simulink model "sistema2020_5"  (R2020b)
settings: Solver=ode15s  StartTime=0.0  StopTime=0.7  MaxStep=1E-2  RelTol=1e-3
libraries: fl_lib x20, ee_lib x12, nesl_utility x12, pid_lib x1
settings Model: LastModifiedBy=josue
settings SolverCC: AlgebraicLoopSolver=LineSearch
settings DataIOCC: SaveOutput=off  SignalLogging=off  DSMLogging=off  ReturnWorkspaceOutputs=off  TimeSaveName=t
settings DebuggingCC: AlgebraicLoopMsg=none  ArtificialAlgebraicLoopMsg=none  MaxConsecutiveZCsMsg=none  UnconnectedInputMsg=none  UnconnectedOutputMsg=none  UnconnectedLineMsg=none  ModelReferenceExtraNoncontSigs=none  OperatingPointInterfaceChecksumMismatchMsg=none
settings ModelReferenceCC: UpdateModelReferenceTargets=IfOutOfDate  EnableRefExpFcnMdlSchedulingChecks=off
settings RTWCC: GPUComputeCapability=5.0

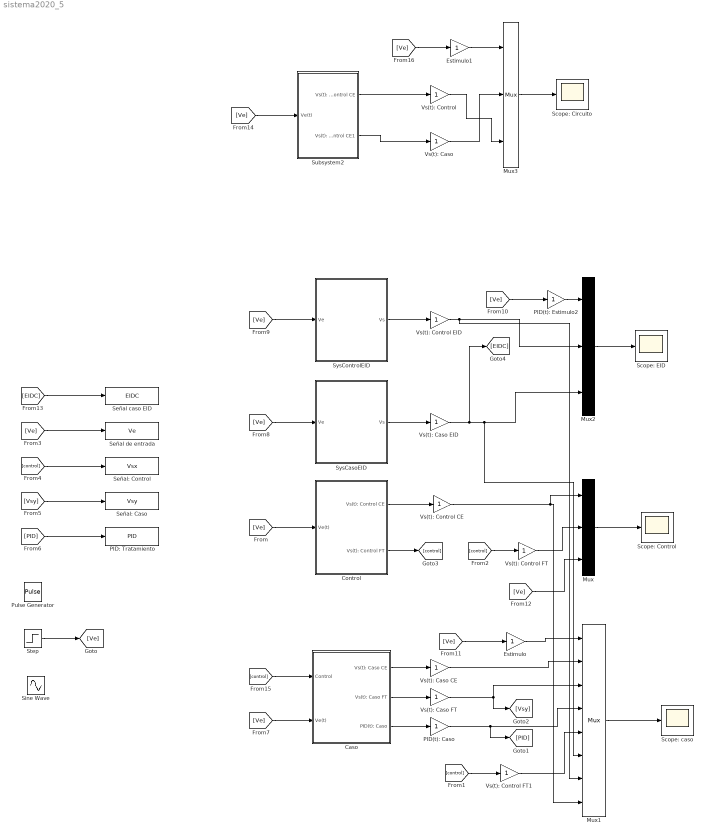
== system sistema2020_5 ==
  Caso : Subsystem
  Control : Subsystem
  Estimulo : Gain
  Estimulo1 : Gain
  Mux : Mux  Inputs=3
  Mux1 : Mux  Inputs=8
  Mux2 : Mux  Inputs=3
  Mux3 : Mux  Inputs=3
  PID(t): Caso : Gain
  PID(t): Estimulo2 : Gain
  PID: Tratamiento : ToWorkspace  VariableName=PID  SampleTime=-1
  Pulse Generator : DiscretePulseGenerator  PulseType=Time based  Period=10  PulseWidth=10  PhaseDelay=1
  Scope: Circuito : Scope
  Scope: Control : Scope
  Scope: EID : Scope
  Scope: caso : Scope
  Señal caso EID : ToWorkspace  VariableName=EIDC  SampleTime=-1
  Señal de entrada : ToWorkspace  VariableName=Ve  SampleTime=-1
  Señal: Caso : ToWorkspace  VariableName=Vsy  SampleTime=-1
  Señal: Control : ToWorkspace  VariableName=Vsx  SampleTime=-1
  Sine Wave : Sin  Frequency=pi/2
  Step : Step  Time=0  Before=1  SampleTime=0
  Subsystem2 : Subsystem
  SysCasoEID : Subsystem
  SysControlEID : Subsystem
  Vs(t): Caso : Gain
  Vs(t): Caso CE : Gain
  "Vs(t): Caso EID " : Gain
  Vs(t): Caso FT : Gain
  Vs(t): Control : Gain
  Vs(t): Control CE : Gain
  Vs(t): Control EID : Gain
  Vs(t): Control FT : Gain
  Vs(t): Control FT1 : Gain
  wires:
  Mux/1 -> Scope: Control/1
  [Ve] -> Control/1(Ve(t))
  Control/1(Vs(t): Control CE) -> Vs(t): Control CE/1
  PID(t): Caso/1 -> [PID], Mux1/4
  Vs(t): Caso CE/1 -> Mux1/2
  Vs(t): Caso FT/1 -> [Vsy], Mux1/3
  Mux1/1 -> Scope: caso/1
  Caso/1(Vs(t): Caso CE) -> Vs(t): Caso CE/1
  Caso/2(Vs(t): Caso FT) -> Vs(t): Caso FT/1
  Caso/3(PID(t): Caso) -> PID(t): Caso/1
  [Ve] -> Caso/2(Ve(t))
  [control] -> Caso/1(Control)
  [control] -> Vs(t): Control FT/1
  Control/2(Vs(t): Control FT) -> [control]
  [PID] -> PID: Tratamiento/1
  [Vsy] -> Señal: Caso/1
  [control] -> Señal: Control/1
  [Ve] -> Señal de entrada/1
  [Ve] -> SysCasoEID/1(Ve)
  Vs(t): Control CE/1 -> Mux1/8, Mux/1
  SysCasoEID/1(Vs) -> "Vs(t): Caso EID "/1
  Vs(t): Control FT/1 -> Mux/2
  [Ve] -> SysControlEID/1(Ve)
  SysControlEID/1(Vs) -> Vs(t): Control EID/1
  Mux2/1 -> Scope: EID/1
  "Vs(t): Caso EID "/1 -> [EIDC], Mux1/6, Mux2/3
  Vs(t): Control EID/1 -> Mux1/7, Mux2/2
  [Ve] -> Mux/3
  [EIDC] -> Señal caso EID/1
  [Ve] -> Subsystem2/1(Ve(t))
  Mux3/1 -> Scope: Circuito/1
  Subsystem2/1(Vs(t): Control CE) -> Vs(t): Control/1
  Subsystem2/2(Vs(t): Control CE1) -> Vs(t): Caso/1
  [Ve] -> Estimulo/1
  Estimulo1/1 -> Mux3/1
  [Ve] -> Estimulo1/1
  Step/1 -> [Ve]
  Vs(t): Caso/1 -> Mux3/2
  Vs(t): Control/1 -> Mux3/3
  [Ve] -> PID(t): Estimulo2/1
  PID(t): Estimulo2/1 -> Mux2/1
  Estimulo/1 -> Mux1/1
  [control] -> Vs(t): Control FT1/1
  Vs(t): Control FT1/1 -> Mux1/5

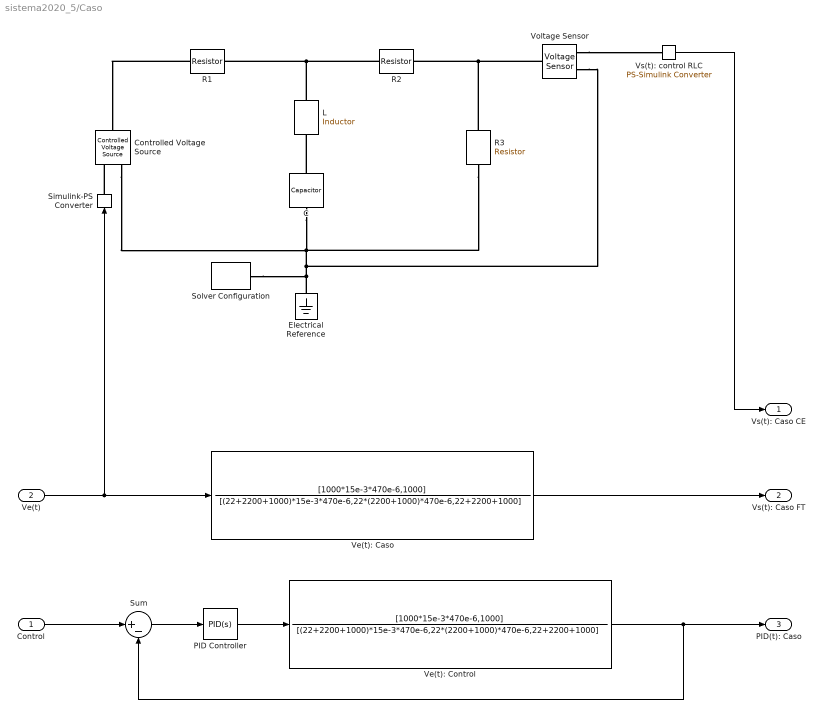
== system sistema2020_5/Caso ==
  Control : Inport
  Ve(t) : Inport  Port=2
  C : fl_lib/Electrical/Electrical Elements/Capacitor  c=470e-6 F  r=1e-6 Ohm  g=0 1/Ohm  i_specify=off  i_priority=None  i=0 A  i_nominal_specify=off  i_nominal_unit=A  i_nominal_value=1  v_specify=off  v_priority=None  v=0 V  v_nominal_specify=off  v_nominal_unit=V  v_nominal_value=1  vc_specify=off  vc_priority=High  vc=0 V  vc_nominal_specify=off  vc_nominal_unit=V  vc_nominal_value=1
  Controlled Voltage Source : fl_lib/Electrical/Electrical Sources/Controlled Voltage Source
  Electrical Reference : fl_lib/Electrical/Electrical Elements/Electrical Reference
  L : fl_lib/Electrical/Electrical Elements/Inductor  l=15e-3 H  r=0 Ohm  g=1e-9 1/Ohm  i_specify=off  i_priority=None  i=0 A  i_nominal_specify=off  i_nominal_unit=A  i_nominal_value=1  v_specify=off  v_priority=None  v=0 V  v_nominal_specify=off  v_nominal_unit=V  v_nominal_value=1  i_L_specify=off  i_L_priority=High  i_L=0 A  i_L_nominal_specify=off  i_L_nominal_unit=A  i_L_nominal_value=1
  PID Controller : pid_lib/PID Controller  Controller=PID  Form=Parallel  TimeDomain=Continuous-time  UseExternalTs=off  SampleTime=-1  IntegratorMethod=Forward Euler  FilterMethod=Forward Euler  ControllerParametersSource=internal  P=34.7718893350657  I=7760.09166130788  D=0.0231467186485559  UseFilter=on  N=113714.226471801  TunerSelectOption=Transfer Function Based (PID Tuner App)  InitialConditionSource=internal  InitialConditionForIntegrator=0  InitialConditionForFilter=0  DifferentiatorICPrevScaledInput=0  ExternalReset=none  TrackingMode=off  Kt=1  LimitOutput=off  SatLimitsSource=internal  UpperSaturationLimit=inf  LowerSaturationLimit=-inf  LinearizeAsGain=on  AntiWindupMode=none  Kb=1  POutMin=[]  POutMax=[]  IOutMin=[]  IOutMax=[]  DOutMin=[]  DOutMax=[]  NOutMin=[]  NOutMax=[]  SumOutMin=[]  SumOutMax=[]  SaturationOutMin=[]  SaturationOutMax=[]  PParamMin=[]  PParamMax=[]  IParamMin=[]  IParamMax=[]  DParamMin=[]  DParamMax=[]  NParamMin=[]  NParamMax=[]  KbParamMin=[]  KbParamMax=[]  KtParamMin=[]  KtParamMax=[]  KbOutMin=[]  KbOutMax=[]  KtOutMin=[]  KtOutMax=[]  IntegratorOutMin=[]  IntegratorOutMax=[]  FilterOutMin=[]  FilterOutMax=[]  SumI1OutMin=[]  SumI1OutMax=[]  SumI2OutMin=[]  SumI2OutMax=[]  SumI3OutMin=[]  SumI3OutMax=[]  SumI4OutMin=[]  SumI4OutMax=[]  SumDOutMin=[]  SumDOutMax=[]  DifferentiatorOutMin=[]  DifferentiatorOutMax=[]  FilterDiffOutCoefMin=[]  FilterDiffOutCoefMax=[]  ReciprocalOutMin=[]  ReciprocalOutMax=[]  SumDenOutMin=[]  SumDenOutMax=[]  SumNumOutMin=[]  SumNumOutMax=[]  DivideOutMin=[]  DivideOutMax=[]  UdiffTsProdOutMin=[]  UdiffTsProdOutMax=[]  NTsProdOutMin=[]  NTsProdOutMax=[]  UintegralTsProdOutMin=[]  UintegralTsProdOutMax=[]  UngainTsProdOutMin=[]  UngainTsProdOutMax=[]  IntegratorContinuousStateAttributes=''  IntegratorStateMustResolveToSignalObject=off  IntegratorRTWStateStorageClass=Auto  FilterContinuousStateAttributes=''  FilterStateMustResolveToSignalObject=off  FilterRTWStateStorageClass=Auto  ParallelPVariant=InternalParameters  IdealPVariant=Disabled  IVariant=InternalParameters  DVariant=InternalParameters  IntegratorVariant=Continuous  SatVariant=Disabled  AWVariant=Passthrough  PCopyVariant=Disabled  TRVariant=Disabled  FdbkBlocksVariant=Forward  IdealPFdbkVariant=Disabled  SatFdbkVariant=Disabled  DerivativeFilterVariant=ContFilter  NVariant=InternalParameters  NCopyVariant=Disabled  FilterICVariant=InternalICsFilter  IntegratorICVariant=InternalICs  ExternalResetVariant=Disabled  TRSumVariant=Passthrough  SumFdbkVariant=Disabled  SumVariant=Sum_PID  TsampFilterVariant=InternalTs  TsampNgainVariant=Passthrough  TsampIntegralVariant=Passthrough  ExternalSaturationOutDataTypeStr=Inherit: Same as second input
  R1 : ee_lib/Passive/Resistor  R=22 Ohm  R_tol=5  enable_R_tol=0  tol_distribution=1  nSigma=4  enable_operating_limits=0  operating_limit_action=2  max_working_voltage=100 V  power_rating=1 W  enable_faults=0  fault_action=1  R_faulted=inf Ohm  enable_temporal_fault=0  t_fault=1 s  enable_behavioral_fault=0  max_permissible_current=1 A  t_fail_on_current=1 s  noise_mode=0  sample_time=1e-3 s  repeatability=1  auto_seed=2645891737  user_seed=0  Tdevice=25 degC  alpha=3.93e-3 1/K  Tmeas=25 degC  thermal_mass=100 J/K  power_derating_T1=70 degC  power_derating_T2=155 degC  operating_temperature_range_vec=[-50, 150] degC  temperature_specify=off  temperature_priority=High  temperature=298.15 K  temperature_nominal_specify=off  temperature_nominal_unit=K  temperature_nominal_value=1
  R2 : ee_lib/Passive/Resistor  R=2200 Ohm  R_tol=5  enable_R_tol=0  tol_distribution=1  nSigma=4  enable_operating_limits=0  operating_limit_action=2  max_working_voltage=100 V  power_rating=1 W  enable_faults=0  fault_action=1  R_faulted=inf Ohm  enable_temporal_fault=0  t_fault=1 s  enable_behavioral_fault=0  max_permissible_current=1 A  t_fail_on_current=1 s  noise_mode=0  sample_time=1e-3 s  repeatability=1  auto_seed=2032760128  user_seed=0  Tdevice=25 degC  alpha=3.93e-3 1/K  Tmeas=25 degC  thermal_mass=100 J/K  power_derating_T1=70 degC  power_derating_T2=155 degC  operating_temperature_range_vec=[-50, 150] degC  temperature_specify=off  temperature_priority=High  temperature=298.15 K  temperature_nominal_specify=off  temperature_nominal_unit=K  temperature_nominal_value=1
  R3 : ee_lib/Passive/Resistor  R=1000 Ohm  R_tol=5  enable_R_tol=0  tol_distribution=1  nSigma=4  enable_operating_limits=0  operating_limit_action=2  max_working_voltage=100 V  power_rating=1 W  enable_faults=0  fault_action=1  R_faulted=inf Ohm  enable_temporal_fault=0  t_fault=1 s  enable_behavioral_fault=0  max_permissible_current=1 A  t_fail_on_current=1 s  noise_mode=0  sample_time=1e-3 s  repeatability=1  auto_seed=1510366082  user_seed=0  Tdevice=25 degC  alpha=3.93e-3 1/K  Tmeas=25 degC  thermal_mass=100 J/K  power_derating_T1=70 degC  power_derating_T2=155 degC  operating_temperature_range_vec=[-50, 150] degC  temperature_specify=off  temperature_priority=High  temperature=298.15 K  temperature_nominal_specify=off  temperature_nominal_unit=K  temperature_nominal_value=1
  Simulink-PS Converter : nesl_utility/Simulink-PS Converter  PhysicalDomain=network_engine_domain  SubClassName=ps_input  LeftPortType=input  RightPortType=output  PseudoPeriodic=off  Frequencies=[]  NoiseDistribution=none  NoiseParameters=[]  Unit=1  AffineConversion=off  FilteringAndDerivatives=provide  SimscapeFilterOrder=1  InputFilterTimeConstant=0.001  UdotUserProvided=0
  Solver Configuration : nesl_utility/Solver Configuration  PhysicalDomain=network_engine_domain  SubClassName=solver  LeftPortType=input  RightPortType=generic  Tones=[]  Harmonics=[]  SimulateNoise=off  Profile=off  UseLocalSampling=off  EnableSwitchedLinearOptims=on  FrequencyDomain=off  UseCCode=off  RelTol=0.001  AbsTol=1e-06  MinStep=1e-09  ToWorkspace=off  RevertToSquareIcSolve=off  NumHomotopyIterations=100  PhasorMode=off  PhasorModeNumHarmonics=1  DoDC=off  ResidualTolerance=1e-09  UseLocalSolver=off  LocalSolverChoice=NE_BACKWARD_EULER_ADVANCER  LocalSolverSampleTime=0.001  DoFixedCost=off  MaxNonlinIter=3  MaxModeIter=2  ComputeImpulses=off  ImpulseIterations=2  LinearAlgebra=auto  EquationFormulation=NE_TIME_EF  DelaysMemoryBudget=1024  AutomaticFiltering=on  FilteringTimeConstant=0.001  PartitionStorageMethod=AS_NEEDED  PartitionMemoryBudget=1024  PartitionMethod=ROBUST
  Sum : Sum  Inputs=|+-
  Ve(t): Caso : TransferFcn  Numerator=[1000*15e-3*470e-6,1000]  Denominator=[(22+2200+1000)*15e-3*470e-6,22*(2200+1000)*470e-6,22+2200+1000]
  Ve(t): Control : TransferFcn  Numerator=[1000*15e-3*470e-6,1000]  Denominator=[(22+2200+1000)*15e-3*470e-6,22*(2200+1000)*470e-6,22+2200+1000]
  Voltage Sensor : fl_lib/Electrical/Electrical Sensors/Voltage Sensor
  "Vs(t): control RLC " : nesl_utility/PS-Simulink Converter  PhysicalDomain=network_engine_domain  SubClassName=ps_output  LeftPortType=input  RightPortType=output  PseudoPeriodic=off  Frequencies=[]  Unit=inherit  AffineConversion=off
  Vs(t): Caso CE : Outport
  Vs(t): Caso FT : Outport  Port=2
  PID(t): Caso : Outport  Port=3
  wires:
  Sum/1 -> PID Controller/1
  PID Controller/1 -> Ve(t): Control/1
  Control/1 -> Sum/1
  Ve(t): Control/1 -> Sum/2, PID(t): Caso/1
  "Vs(t): control RLC "/1 -> Vs(t): Caso CE/1
  Ve(t): Caso/1 -> Vs(t): Caso FT/1
  Ve(t)/1 -> Ve(t): Caso/1, Simulink-PS Converter/1
  connections:
  C/RConn1 -- Voltage Sensor/RConn2 -- Solver Configuration/RConn1 -- Electrical Reference/LConn1 -- R3/RConn1 -- Controlled Voltage Source/RConn2
  R1/RConn1 -- R2/LConn1 -- L/LConn1
  Voltage Sensor/LConn1 -- R3/LConn1 -- R2/RConn1
  Voltage Sensor/RConn1 -- "Vs(t): control RLC "/LConn1
  C/LConn1 -- L/RConn1
  Simulink-PS Converter/RConn1 -- Controlled Voltage Source/RConn1
  R1/LConn1 -- Controlled Voltage Source/LConn1

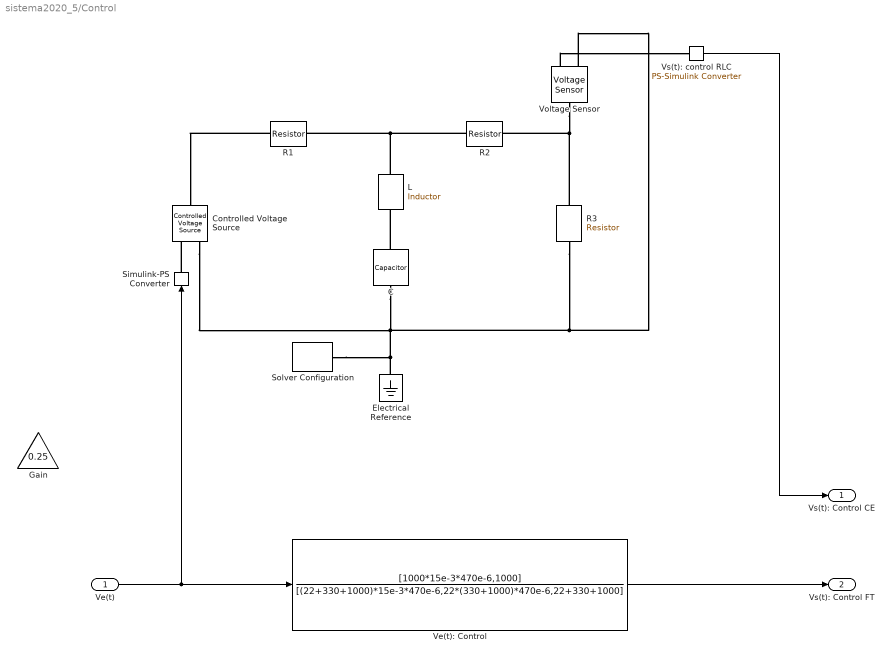
== system sistema2020_5/Control ==
  Ve(t) : Inport
  C : fl_lib/Electrical/Electrical Elements/Capacitor  c=470e-6 F  r=1e-6 Ohm  g=0 1/Ohm  i_specify=off  i_priority=None  i=0 A  i_nominal_specify=off  i_nominal_unit=A  i_nominal_value=1  v_specify=off  v_priority=None  v=0 V  v_nominal_specify=off  v_nominal_unit=V  v_nominal_value=1  vc_specify=off  vc_priority=High  vc=0 V  vc_nominal_specify=off  vc_nominal_unit=V  vc_nominal_value=1
  Controlled Voltage Source : fl_lib/Electrical/Electrical Sources/Controlled Voltage Source
  Electrical Reference : fl_lib/Electrical/Electrical Elements/Electrical Reference
  Gain : Gain  Gain=0.25
  L : fl_lib/Electrical/Electrical Elements/Inductor  l=15e-3 H  r=0 Ohm  g=1e-9 1/Ohm  i_specify=off  i_priority=None  i=0 A  i_nominal_specify=off  i_nominal_unit=A  i_nominal_value=1  v_specify=off  v_priority=None  v=0 V  v_nominal_specify=off  v_nominal_unit=V  v_nominal_value=1  i_L_specify=off  i_L_priority=High  i_L=0 A  i_L_nominal_specify=off  i_L_nominal_unit=A  i_L_nominal_value=1
  R1 : ee_lib/Passive/Resistor  R=22 Ohm  R_tol=5  enable_R_tol=0  tol_distribution=1  nSigma=4  enable_operating_limits=0  operating_limit_action=2  max_working_voltage=100 V  power_rating=1 W  enable_faults=0  fault_action=1  R_faulted=inf Ohm  enable_temporal_fault=0  t_fault=1 s  enable_behavioral_fault=0  max_permissible_current=1 A  t_fail_on_current=1 s  noise_mode=0  sample_time=1e-3 s  repeatability=1  auto_seed=1196140742  user_seed=0  Tdevice=25 degC  alpha=3.93e-3 1/K  Tmeas=25 degC  thermal_mass=100 J/K  power_derating_T1=70 degC  power_derating_T2=155 degC  operating_temperature_range_vec=[-50, 150] degC  temperature_specify=off  temperature_priority=High  temperature=298.15 K  temperature_nominal_specify=off  temperature_nominal_unit=K  temperature_nominal_value=1
  R2 : ee_lib/Passive/Resistor  R=330 Ohm  R_tol=5  enable_R_tol=0  tol_distribution=1  nSigma=4  enable_operating_limits=0  operating_limit_action=2  max_working_voltage=100 V  power_rating=1 W  enable_faults=0  fault_action=1  R_faulted=inf Ohm  enable_temporal_fault=0  t_fault=1 s  enable_behavioral_fault=0  max_permissible_current=1 A  t_fail_on_current=1 s  noise_mode=0  sample_time=1e-3 s  repeatability=1  auto_seed=2348838240  user_seed=0  Tdevice=25 degC  alpha=3.93e-3 1/K  Tmeas=25 degC  thermal_mass=100 J/K  power_derating_T1=70 degC  power_derating_T2=155 degC  operating_temperature_range_vec=[-50, 150] degC  temperature_specify=off  temperature_priority=High  temperature=298.15 K  temperature_nominal_specify=off  temperature_nominal_unit=K  temperature_nominal_value=1
  R3 : ee_lib/Passive/Resistor  R=1000 Ohm  R_tol=5  enable_R_tol=0  tol_distribution=1  nSigma=4  enable_operating_limits=0  operating_limit_action=2  max_working_voltage=100 V  power_rating=1 W  enable_faults=0  fault_action=1  R_faulted=inf Ohm  enable_temporal_fault=0  t_fault=1 s  enable_behavioral_fault=0  max_permissible_current=1 A  t_fail_on_current=1 s  noise_mode=0  sample_time=1e-3 s  repeatability=1  auto_seed=4112460543  user_seed=0  Tdevice=25 degC  alpha=3.93e-3 1/K  Tmeas=25 degC  thermal_mass=100 J/K  power_derating_T1=70 degC  power_derating_T2=155 degC  operating_temperature_range_vec=[-50, 150] degC  temperature_specify=off  temperature_priority=High  temperature=298.15 K  temperature_nominal_specify=off  temperature_nominal_unit=K  temperature_nominal_value=1
  Simulink-PS Converter : nesl_utility/Simulink-PS Converter  PhysicalDomain=network_engine_domain  SubClassName=ps_input  LeftPortType=input  RightPortType=output  PseudoPeriodic=off  Frequencies=[]  NoiseDistribution=none  NoiseParameters=[]  Unit=1  AffineConversion=off  FilteringAndDerivatives=provide  SimscapeFilterOrder=1  InputFilterTimeConstant=0.001  UdotUserProvided=0
  Solver Configuration : nesl_utility/Solver Configuration  PhysicalDomain=network_engine_domain  SubClassName=solver  LeftPortType=input  RightPortType=generic  Tones=[]  Harmonics=[]  SimulateNoise=off  Profile=off  UseLocalSampling=off  EnableSwitchedLinearOptims=on  FrequencyDomain=off  UseCCode=off  RelTol=0.001  AbsTol=1e-06  MinStep=1e-09  ToWorkspace=off  RevertToSquareIcSolve=off  NumHomotopyIterations=100  PhasorMode=off  PhasorModeNumHarmonics=1  DoDC=off  ResidualTolerance=1e-09  UseLocalSolver=off  LocalSolverChoice=NE_BACKWARD_EULER_ADVANCER  LocalSolverSampleTime=0.001  DoFixedCost=off  MaxNonlinIter=3  MaxModeIter=2  ComputeImpulses=off  ImpulseIterations=2  LinearAlgebra=auto  EquationFormulation=NE_TIME_EF  DelaysMemoryBudget=1024  AutomaticFiltering=on  FilteringTimeConstant=0.001  PartitionStorageMethod=AS_NEEDED  PartitionMemoryBudget=1024  PartitionMethod=ROBUST
  Ve(t): Control : TransferFcn  Numerator=[1000*15e-3*470e-6,1000]  Denominator=[(22+330+1000)*15e-3*470e-6,22*(330+1000)*470e-6,22+330+1000]
  Voltage Sensor : fl_lib/Electrical/Electrical Sensors/Voltage Sensor
  "Vs(t): control RLC " : nesl_utility/PS-Simulink Converter  PhysicalDomain=network_engine_domain  SubClassName=ps_output  LeftPortType=input  RightPortType=output  PseudoPeriodic=off  Frequencies=[]  Unit=inherit  AffineConversion=off
  Vs(t): Control CE : Outport
  Vs(t): Control FT : Outport  Port=2
  wires:
  Ve(t): Control/1 -> Vs(t): Control FT/1
  Ve(t)/1 -> Ve(t): Control/1, Simulink-PS Converter/1
  "Vs(t): control RLC "/1 -> Vs(t): Control CE/1
  connections:
  Voltage Sensor/LConn1 -- R3/LConn1 -- R2/RConn1
  C/RConn1 -- Voltage Sensor/RConn2 -- R3/RConn1 -- Controlled Voltage Source/RConn2 -- Solver Configuration/RConn1 -- Electrical Reference/LConn1
  R1/RConn1 -- R2/LConn1 -- L/LConn1
  Simulink-PS Converter/RConn1 -- Controlled Voltage Source/RConn1
  R1/LConn1 -- Controlled Voltage Source/LConn1
  Voltage Sensor/RConn1 -- "Vs(t): control RLC "/LConn1
  C/LConn1 -- L/RConn1

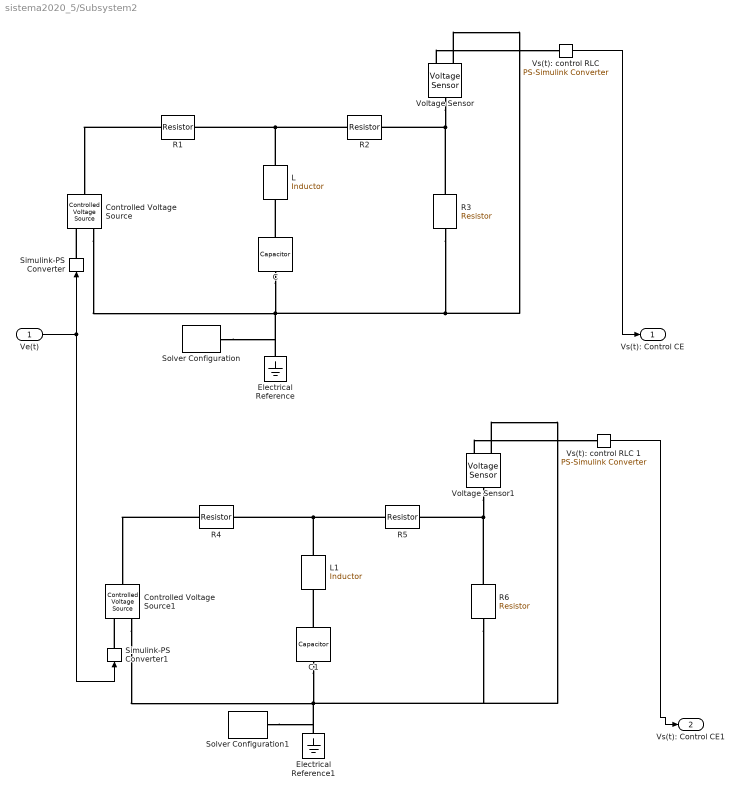
== system sistema2020_5/Subsystem2 ==
  Ve(t) : Inport
  C : fl_lib/Electrical/Electrical Elements/Capacitor  c=470e-6 F  r=1e-6 Ohm  g=0 1/Ohm  i_specify=off  i_priority=None  i=0 A  i_nominal_specify=off  i_nominal_unit=A  i_nominal_value=1  v_specify=off  v_priority=None  v=0 V  v_nominal_specify=off  v_nominal_unit=V  v_nominal_value=1  vc_specify=off  vc_priority=High  vc=0 V  vc_nominal_specify=off  vc_nominal_unit=V  vc_nominal_value=1
  C1 : fl_lib/Electrical/Electrical Elements/Capacitor  c=470e-6 F  r=1e-6 Ohm  g=0 1/Ohm  i_specify=off  i_priority=None  i=0 A  i_nominal_specify=off  i_nominal_unit=A  i_nominal_value=1  v_specify=off  v_priority=None  v=0 V  v_nominal_specify=off  v_nominal_unit=V  v_nominal_value=1  vc_specify=off  vc_priority=High  vc=0 V  vc_nominal_specify=off  vc_nominal_unit=V  vc_nominal_value=1
  Controlled Voltage Source : fl_lib/Electrical/Electrical Sources/Controlled Voltage Source
  Controlled Voltage Source1 : fl_lib/Electrical/Electrical Sources/Controlled Voltage Source
  Electrical Reference : fl_lib/Electrical/Electrical Elements/Electrical Reference
  Electrical Reference1 : fl_lib/Electrical/Electrical Elements/Electrical Reference
  L : fl_lib/Electrical/Electrical Elements/Inductor  l=15e-3 H  r=0 Ohm  g=1e-9 1/Ohm  i_specify=off  i_priority=None  i=0 A  i_nominal_specify=off  i_nominal_unit=A  i_nominal_value=1  v_specify=off  v_priority=None  v=0 V  v_nominal_specify=off  v_nominal_unit=V  v_nominal_value=1  i_L_specify=off  i_L_priority=High  i_L=0 A  i_L_nominal_specify=off  i_L_nominal_unit=A  i_L_nominal_value=1
  L1 : fl_lib/Electrical/Electrical Elements/Inductor  l=15e-3 H  r=0 Ohm  g=1e-9 1/Ohm  i_specify=off  i_priority=None  i=0 A  i_nominal_specify=off  i_nominal_unit=A  i_nominal_value=1  v_specify=off  v_priority=None  v=0 V  v_nominal_specify=off  v_nominal_unit=V  v_nominal_value=1  i_L_specify=off  i_L_priority=High  i_L=0 A  i_L_nominal_specify=off  i_L_nominal_unit=A  i_L_nominal_value=1
  R1 : ee_lib/Passive/Resistor  R=22 Ohm  R_tol=5  enable_R_tol=0  tol_distribution=1  nSigma=4  enable_operating_limits=0  operating_limit_action=2  max_working_voltage=100 V  power_rating=1 W  enable_faults=0  fault_action=1  R_faulted=inf Ohm  enable_temporal_fault=0  t_fault=1 s  enable_behavioral_fault=0  max_permissible_current=1 A  t_fail_on_current=1 s  noise_mode=0  sample_time=1e-3 s  repeatability=1  auto_seed=386335224  user_seed=0  Tdevice=25 degC  alpha=3.93e-3 1/K  Tmeas=25 degC  thermal_mass=100 J/K  power_derating_T1=70 degC  power_derating_T2=155 degC  operating_temperature_range_vec=[-50, 150] degC  temperature_specify=off  temperature_priority=High  temperature=298.15 K  temperature_nominal_specify=off  temperature_nominal_unit=K  temperature_nominal_value=1
  R2 : ee_lib/Passive/Resistor  R=330 Ohm  R_tol=5  enable_R_tol=0  tol_distribution=1  nSigma=4  enable_operating_limits=0  operating_limit_action=2  max_working_voltage=100 V  power_rating=1 W  enable_faults=0  fault_action=1  R_faulted=inf Ohm  enable_temporal_fault=0  t_fault=1 s  enable_behavioral_fault=0  max_permissible_current=1 A  t_fail_on_current=1 s  noise_mode=0  sample_time=1e-3 s  repeatability=1  auto_seed=3499211588  user_seed=0  Tdevice=25 degC  alpha=3.93e-3 1/K  Tmeas=25 degC  thermal_mass=100 J/K  power_derating_T1=70 degC  power_derating_T2=155 degC  operating_temperature_range_vec=[-50, 150] degC  temperature_specify=off  temperature_priority=High  temperature=298.15 K  temperature_nominal_specify=off  temperature_nominal_unit=K  temperature_nominal_value=1
  R3 : ee_lib/Passive/Resistor  R=1000 Ohm  R_tol=5  enable_R_tol=0  tol_distribution=1  nSigma=4  enable_operating_limits=0  operating_limit_action=2  max_working_voltage=100 V  power_rating=1 W  enable_faults=0  fault_action=1  R_faulted=inf Ohm  enable_temporal_fault=0  t_fault=1 s  enable_behavioral_fault=0  max_permissible_current=1 A  t_fail_on_current=1 s  noise_mode=0  sample_time=1e-3 s  repeatability=1  auto_seed=1943870165  user_seed=0  Tdevice=25 degC  alpha=3.93e-3 1/K  Tmeas=25 degC  thermal_mass=100 J/K  power_derating_T1=70 degC  power_derating_T2=155 degC  operating_temperature_range_vec=[-50, 150] degC  temperature_specify=off  temperature_priority=High  temperature=298.15 K  temperature_nominal_specify=off  temperature_nominal_unit=K  temperature_nominal_value=1
  R4 : ee_lib/Passive/Resistor  R=22 Ohm  R_tol=5  enable_R_tol=0  tol_distribution=1  nSigma=4  enable_operating_limits=0  operating_limit_action=2  max_working_voltage=100 V  power_rating=1 W  enable_faults=0  fault_action=1  R_faulted=inf Ohm  enable_temporal_fault=0  t_fault=1 s  enable_behavioral_fault=0  max_permissible_current=1 A  t_fail_on_current=1 s  noise_mode=0  sample_time=1e-3 s  repeatability=1  auto_seed=2874086048  user_seed=0  Tdevice=25 degC  alpha=3.93e-3 1/K  Tmeas=25 degC  thermal_mass=100 J/K  power_derating_T1=70 degC  power_derating_T2=155 degC  operating_temperature_range_vec=[-50, 150] degC  temperature_specify=off  temperature_priority=High  temperature=298.15 K  temperature_nominal_specify=off  temperature_nominal_unit=K  temperature_nominal_value=1
  R5 : ee_lib/Passive/Resistor  R=3300 Ohm  R_tol=5  enable_R_tol=0  tol_distribution=1  nSigma=4  enable_operating_limits=0  operating_limit_action=2  max_working_voltage=100 V  power_rating=1 W  enable_faults=0  fault_action=1  R_faulted=inf Ohm  enable_temporal_fault=0  t_fault=1 s  enable_behavioral_fault=0  max_permissible_current=1 A  t_fail_on_current=1 s  noise_mode=0  sample_time=1e-3 s  repeatability=1  auto_seed=817904655  user_seed=0  Tdevice=25 degC  alpha=3.93e-3 1/K  Tmeas=25 degC  thermal_mass=100 J/K  power_derating_T1=70 degC  power_derating_T2=155 degC  operating_temperature_range_vec=[-50, 150] degC  temperature_specify=off  temperature_priority=High  temperature=298.15 K  temperature_nominal_specify=off  temperature_nominal_unit=K  temperature_nominal_value=1
  R6 : ee_lib/Passive/Resistor  R=1000 Ohm  R_tol=5  enable_R_tol=0  tol_distribution=1  nSigma=4  enable_operating_limits=0  operating_limit_action=2  max_working_voltage=100 V  power_rating=1 W  enable_faults=0  fault_action=1  R_faulted=inf Ohm  enable_temporal_fault=0  t_fault=1 s  enable_behavioral_fault=0  max_permissible_current=1 A  t_fail_on_current=1 s  noise_mode=0  sample_time=1e-3 s  repeatability=1  auto_seed=1584484500  user_seed=0  Tdevice=25 degC  alpha=3.93e-3 1/K  Tmeas=25 degC  thermal_mass=100 J/K  power_derating_T1=70 degC  power_derating_T2=155 degC  operating_temperature_range_vec=[-50, 150] degC  temperature_specify=off  temperature_priority=High  temperature=298.15 K  temperature_nominal_specify=off  temperature_nominal_unit=K  temperature_nominal_value=1
  Simulink-PS Converter : nesl_utility/Simulink-PS Converter  PhysicalDomain=network_engine_domain  SubClassName=ps_input  LeftPortType=input  RightPortType=output  PseudoPeriodic=off  Frequencies=[]  NoiseDistribution=none  NoiseParameters=[]  Unit=1  AffineConversion=off  FilteringAndDerivatives=provide  SimscapeFilterOrder=1  InputFilterTimeConstant=0.001  UdotUserProvided=0
  Simulink-PS Converter1 : nesl_utility/Simulink-PS Converter  PhysicalDomain=network_engine_domain  SubClassName=ps_input  LeftPortType=input  RightPortType=output  PseudoPeriodic=off  Frequencies=[]  NoiseDistribution=none  NoiseParameters=[]  Unit=1  AffineConversion=off  FilteringAndDerivatives=provide  SimscapeFilterOrder=1  InputFilterTimeConstant=0.001  UdotUserProvided=0
  Solver Configuration : nesl_utility/Solver Configuration  PhysicalDomain=network_engine_domain  SubClassName=solver  LeftPortType=input  RightPortType=generic  Tones=[]  Harmonics=[]  SimulateNoise=off  Profile=off  UseLocalSampling=off  EnableSwitchedLinearOptims=on  FrequencyDomain=off  UseCCode=off  RelTol=0.001  AbsTol=1e-06  MinStep=1e-09  ToWorkspace=off  RevertToSquareIcSolve=off  NumHomotopyIterations=100  PhasorMode=off  PhasorModeNumHarmonics=1  DoDC=off  ResidualTolerance=1e-09  UseLocalSolver=off  LocalSolverChoice=NE_BACKWARD_EULER_ADVANCER  LocalSolverSampleTime=0.001  DoFixedCost=off  MaxNonlinIter=3  MaxModeIter=2  ComputeImpulses=off  ImpulseIterations=2  LinearAlgebra=auto  EquationFormulation=NE_TIME_EF  DelaysMemoryBudget=1024  AutomaticFiltering=on  FilteringTimeConstant=0.001  PartitionStorageMethod=AS_NEEDED  PartitionMemoryBudget=1024  PartitionMethod=ROBUST
  Solver Configuration1 : nesl_utility/Solver Configuration  PhysicalDomain=network_engine_domain  SubClassName=solver  LeftPortType=input  RightPortType=generic  Tones=[]  Harmonics=[]  SimulateNoise=off  Profile=off  UseLocalSampling=off  EnableSwitchedLinearOptims=on  FrequencyDomain=off  UseCCode=off  RelTol=0.001  AbsTol=1e-06  MinStep=1e-09  ToWorkspace=off  RevertToSquareIcSolve=off  NumHomotopyIterations=100  PhasorMode=off  PhasorModeNumHarmonics=1  DoDC=off  ResidualTolerance=1e-09  UseLocalSolver=off  LocalSolverChoice=NE_BACKWARD_EULER_ADVANCER  LocalSolverSampleTime=0.001  DoFixedCost=off  MaxNonlinIter=3  MaxModeIter=2  ComputeImpulses=off  ImpulseIterations=2  LinearAlgebra=auto  EquationFormulation=NE_TIME_EF  DelaysMemoryBudget=1024  AutomaticFiltering=on  FilteringTimeConstant=0.001  PartitionStorageMethod=AS_NEEDED  PartitionMemoryBudget=1024  PartitionMethod=ROBUST
  Voltage Sensor : fl_lib/Electrical/Electrical Sensors/Voltage Sensor
  Voltage Sensor1 : fl_lib/Electrical/Electrical Sensors/Voltage Sensor
  "Vs(t): control RLC " : nesl_utility/PS-Simulink Converter  PhysicalDomain=network_engine_domain  SubClassName=ps_output  LeftPortType=input  RightPortType=output  PseudoPeriodic=off  Frequencies=[]  Unit=inherit  AffineConversion=off
  Vs(t): control RLC 1 : nesl_utility/PS-Simulink Converter  PhysicalDomain=network_engine_domain  SubClassName=ps_output  LeftPortType=input  RightPortType=output  PseudoPeriodic=off  Frequencies=[]  Unit=inherit  AffineConversion=off
  Vs(t): Control CE : Outport
  Vs(t): Control CE1 : Outport  Port=2
  wires:
  Ve(t)/1 -> Simulink-PS Converter/1, Simulink-PS Converter1/1
  "Vs(t): control RLC "/1 -> Vs(t): Control CE/1
  Vs(t): control RLC 1/1 -> Vs(t): Control CE1/1
  connections:
  Voltage Sensor/RConn2 -- Controlled Voltage Source/RConn2 -- Solver Configuration/RConn1 -- Electrical Reference/LConn1 -- C/RConn1 -- R3/RConn1
  Voltage Sensor/RConn1 -- "Vs(t): control RLC "/LConn1
  Simulink-PS Converter/RConn1 -- Controlled Voltage Source/RConn1
  R1/LConn1 -- Controlled Voltage Source/LConn1
  R2/LConn1 -- L/LConn1 -- R1/RConn1
  C/LConn1 -- L/RConn1
  R3/LConn1 -- R2/RConn1 -- Voltage Sensor/LConn1
  C1/RConn1 -- Solver Configuration1/RConn1 -- Electrical Reference1/LConn1 -- Controlled Voltage Source1/RConn2 -- R6/RConn1 -- Voltage Sensor1/RConn2
  R5/LConn1 -- L1/LConn1 -- R4/RConn1
  Voltage Sensor1/LConn1 -- R5/RConn1 -- R6/LConn1
  Simulink-PS Converter1/RConn1 -- Controlled Voltage Source1/RConn1
  Voltage Sensor1/RConn1 -- Vs(t): control RLC 1/LConn1
  R4/LConn1 -- Controlled Voltage Source1/LConn1
  C1/LConn1 -- L1/RConn1

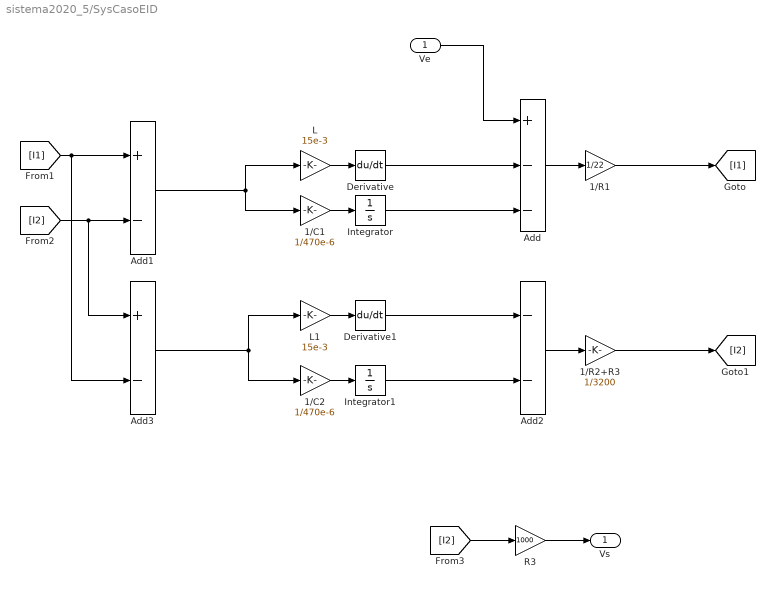
== system sistema2020_5/SysCasoEID ==
  Ve : Inport
  1/C1 : Gain  Gain=1/470e-6
  1/C2 : Gain  Gain=1/470e-6
  1/R1 : Gain  Gain=1/22
  1/R2+R3 : Gain  Gain=1/3200
  Add : Sum  Inputs=+--
  Add1 : Sum  Inputs=+-
  Add2 : Sum  Inputs=--
  Add3 : Sum  Inputs=+-
  Derivative : Derivative
  Derivative1 : Derivative
  Integrator : Integrator
  Integrator1 : Integrator
  L : Gain  Gain=15e-3
  L1 : Gain  Gain=15e-3
  R3 : Gain  Gain=1000
  Vs : Outport
  wires:
  Derivative1/1 -> Add2/1
  L/1 -> Derivative/1
  1/R1/1 -> [I1]
  R3/1 -> Vs/1
  1/C1/1 -> Integrator/1
  1/R2+R3/1 -> [I2]
  Integrator/1 -> Add/3
  Integrator1/1 -> Add2/2
  Add/1 -> 1/R1/1
  [I2] -> R3/1
  1/C2/1 -> Integrator1/1
  Add1/1 -> 1/C1/1, L/1
  Ve/1 -> Add/1
  Add2/1 -> 1/R2+R3/1
  L1/1 -> Derivative1/1
  Add3/1 -> L1/1, 1/C2/1
  [I1] -> Add3/2, Add1/1
  Derivative/1 -> Add/2
  [I2] -> Add3/1, Add1/2

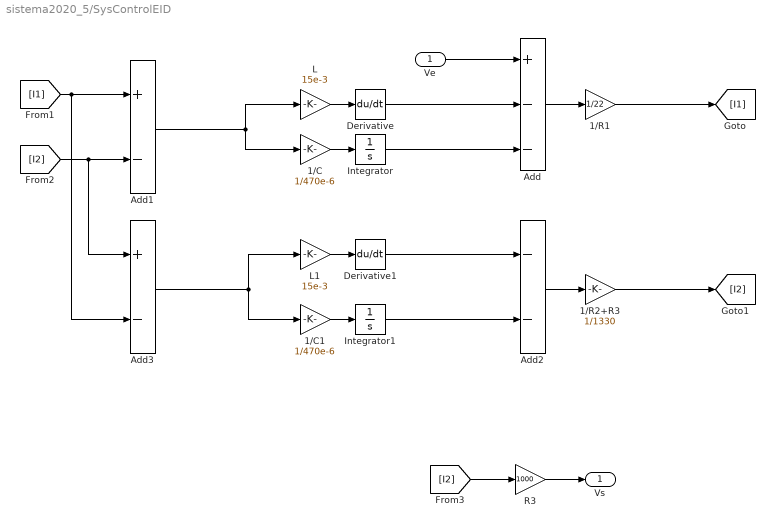
== system sistema2020_5/SysControlEID ==
  Ve : Inport
  1/C : Gain  Gain=1/470e-6
  1/C1 : Gain  Gain=1/470e-6
  1/R1 : Gain  Gain=1/22
  1/R2+R3 : Gain  Gain=1/1330
  Add : Sum  Inputs=+--
  Add1 : Sum  Inputs=+-
  Add2 : Sum  Inputs=--
  Add3 : Sum  Inputs=+-
  Derivative : Derivative
  Derivative1 : Derivative
  Integrator : Integrator
  Integrator1 : Integrator
  L : Gain  Gain=15e-3
  L1 : Gain  Gain=15e-3
  R3 : Gain  Gain=1000
  Vs : Outport
  wires:
  Ve/1 -> Add/1
  L/1 -> Derivative/1
  1/C/1 -> Integrator/1
  Integrator/1 -> Add/3
  Derivative/1 -> Add/2
  1/R1/1 -> [I1]
  Add/1 -> 1/R1/1
  [I1] -> Add3/2, Add1/1
  [I2] -> Add3/1, Add1/2
  Add1/1 -> 1/C/1, L/1
  1/C1/1 -> Integrator1/1
  L1/1 -> Derivative1/1
  Integrator1/1 -> Add2/2
  Derivative1/1 -> Add2/1
  Add3/1 -> L1/1, 1/C1/1
  Add2/1 -> 1/R2+R3/1
  1/R2+R3/1 -> [I2]
  [I2] -> R3/1
  R3/1 -> Vs/1
